simulink model "Morimoto1990_FieldWeakening"  (R2024b)
settings: Solver=FixedStepDiscrete  StartTime=0.0  StopTime=Duration  FixedStep=h  RelTol=1e-3
InitFcn:
  | demoModel=bdroot; demoWorkspace=get_param(demoModel,'ModelWorkspace');
  | demoCases=getVariable(demoWorkspace,'DemoCases');
  | demoCaseName=get_param([demoModel '/Experiment_Settings'],'CaseName');
  | demoSelected=find(strcmp(demoCaseName,{demoCases.name}),1);
  | demoValues=demoCases(demoSelected).variables; demoNames=fieldnames(demoValues);
  | for demoIndex=1:numel(demoNames), assignin(demoWorkspace,demoNames{demoIndex},demoValues.(demoNames{demoIndex})); end
  | clear demoModel demoWorkspace demoCases demoCaseName demoSelected demoValues demoNames demoIndex;
model workspace (MAT data in the model file):
  DemoCases : object (value not decoded)
  SpeedProgram = [0  0; 0.22  900; 0.34  900; 0.95  4200; 1.65  4200]
  UseWeakening = 1
values from neighbouring files (symbols this model uses):
  B = 0.0002    [Morimoto1990_FieldWeakening.sldd]
  BaseCap = 11.4197598 11.4197598 11.4197598 11.4197598 11.4197598 11.4197598 11.4197598 11.4197598 11.4197598 11.4197598 11.4197598 11.4197598 11.4197598 11.4197598 11.4197598 11.4197598 11.4197598 11.4197598 11.4197598 11.4197598 11.4197598 11.4197598 11.4197598 11.4197598 11.4197598 11.4197598 11.4197598 11.4197598 11.4197598 11.4197598 11.4197598 11.4197598 11.4197598 11.4197598 11.4197598 11.4197598 11.4    [Morimoto1990_FieldWeakening.sldd]
  BaseId = -0.0 -0.0 -0.0 -0.0 -0.0 -0.0 -0.0 -0.0 -0.0 -0.0 -0.0 -0.0 -0.0 -0.0 -0.0 -0.0 -0.0 -0.0 -0.0 -0.0 -0.0 -0.0 -0.0 -0.0 -0.0 -0.0 -0.0 -0.0 -0.0 -0.0 -0.0 -0.0 -0.0 -0.0 -0.0 -0.0 -0.0 -0.0 -0.0 -0.0 -0.0 -0.0 -0.0 -0.0 -0.0 -0.0 -0.0 -0.0 -0.0 -0.0 -0.0 -0.0 -0.0 -0.0 -0.0 -0.0 -0.0 -0.0 -0.0 -0.0 -0.0 -0.0 -0.0 -0.0 -0.0 -0.0 -0.0 -0.0 -0.0 -0.0 -0.0 -0.0 -0.0 -0.0 -0.0 -0.0 -0.0 -0.0 -0.0 -0.0    [Morimoto1990_FieldWeakening.sldd]
  BaseIq = 0.0 0.0 0.0 0.0 0.0 0.0 0.0 0.0 0.0 0.0 0.0 0.0 0.0 0.0 0.0 0.0 0.0 0.0 0.0 0.0 0.0 0.0 0.0 0.0 0.0 0.0 0.0 0.0 0.0 0.0 0.0 0.0 0.0 0.0 0.0 0.0 0.0 0.0 0.0 0.0 0.0 0.0 0.0 0.0 0.0 0.0 0.0 0.0 0.0 0.0 0.0 0.0 0.0 0.0 0.0 0.0 0.0 0.0 0.0 0.0 0.0 0.0 0.0 0.0 0.0 0.0 0.0 0.0 0.0 0.0 0.0 0.0 0.0 0.0 0.0 0.0 0.0 0.0 0.0 0.0 0.0 0.0 0.0 0.0 0.0 0.0 0.0 0.0 0.0 0.0 0.0 0.0 0.0 0.0 0.0 0.0 0.0 0.0 0.0 0.0    [Morimoto1990_FieldWeakening.sldd]
  BusReadyRatio = 0.94    [Morimoto1990_FieldWeakening.sldd]
  CurrentBandwidth = 1450.0    [Morimoto1990_FieldWeakening.sldd]
  CurrentKaw = 1500.0    [Morimoto1990_FieldWeakening.sldd]
  EnableThreshold = 0.5    [Morimoto1990_FieldWeakening.sldd]
  Fraction = 0.0 0.025 0.05 0.075 0.1 0.125 0.15 0.175 0.2 0.225 0.25 0.275 0.3 0.325 0.35 0.375 0.4 0.425 0.45 0.475 0.5 0.525 0.55 0.575 0.6 0.625 0.65 0.675 0.7 0.725 0.75 0.775 0.8 0.825 0.85 0.875 0.9 0.925 0.95 0.975 1.0    [Morimoto1990_FieldWeakening.sldd]
  FwCap = 11.4197598 11.4197598 11.4197598 11.4197598 11.4197598 11.4197598 11.4197598 11.4197598 11.4197598 11.4197598 11.4197598 11.4197598 11.4197598 11.4197598 11.4197598 11.4197598 11.4197598 11.4197598 11.4197598 11.4197598 11.4197598 11.4197598 11.4197598 11.4197598 11.4197598 11.4197598 11.4197598 11.4197598 11.4197598 11.4197598 11.4197598 11.4197598 11.4197598 11.4197598 11.4197598 11.4197598 11.4    [Morimoto1990_FieldWeakening.sldd]
  FwId = -0.0 -0.0 -0.0 -0.0 -0.0 -0.0 -0.0 -0.0 -0.0 -0.0 -0.0 -0.0 -0.0 -0.0 -0.0 -0.0 -0.0 -0.0 -0.0 -0.0 -0.0 -0.0 -0.0 -0.0 -0.0 -0.0 -0.0 -0.0 -0.0 -0.0 -0.0 -0.0 -0.0 -0.0 -0.0 -0.0 -0.0 -0.0 -0.0 -0.0 -0.0 -0.0 -0.0 -0.0 -0.0 -0.0 -0.0 -0.0 -0.0 -0.0 -0.0 -0.0 -0.0 -0.0 -0.0 -0.0 -0.0 -0.0 -0.0 -0.0 -0.0 -0.0 -0.0 -0.0 -0.0 -0.0 -0.0 -0.0 -0.0 -0.0 -0.0 -0.0 -0.0 -0.0 -0.0 -0.0 -0.0 -0.0 -0.0 -0.0    [Morimoto1990_FieldWeakening.sldd]
  FwIq = 0.0 0.0 0.0 0.0 0.0 0.0 0.0 0.0 0.0 0.0 0.0 0.0 0.0 0.0 0.0 0.0 0.0 0.0 0.0 0.0 0.0 0.0 0.0 0.0 0.0 0.0 0.0 0.0 0.0 0.0 0.0 0.0 0.0 0.0 0.0 0.0 0.0 0.0 0.0 0.0 0.0 0.0 0.0 0.0 0.0 0.0 0.0 0.0 0.0 0.0 0.0 0.0 0.0 0.0 0.0 0.0 0.0 0.0 0.0 0.0 0.0 0.0 0.0 0.0 0.0 0.0 0.0 0.0 0.0 0.0 0.0 0.0 0.0 0.0 0.0 0.0 0.0 0.0 0.0 0.0 0.0 0.0 0.0 0.0 0.0 0.0 0.0 0.0 0.0 0.0 0.0 0.0 0.0 0.0 0.0 0.0 0.0 0.0 0.0 0.0    [Morimoto1990_FieldWeakening.sldd]
  h = 2.5E-6    [Morimoto1990_FieldWeakening.sldd]
  J = 0.0006    [Morimoto1990_FieldWeakening.sldd]
  Ld = 0.001875    [Morimoto1990_FieldWeakening.sldd]
  Lq = 0.00375    [Morimoto1990_FieldWeakening.sldd]
  Ngrid = 0.0 25.0 50.0 75.0 100.0 125.0 150.0 175.0 200.0 225.0 250.0 275.0 300.0 325.0 350.0 375.0 400.0 425.0 450.0 475.0 500.0 525.0 550.0 575.0 600.0 625.0 650.0 675.0 700.0 725.0 750.0 775.0 800.0 825.0 850.0 875.0 900.0 925.0 950.0 975.0 1000.0 1025.0 1050.0 1075.0 1100.0 1125.0 1150.0 1175.0 1200.0 1225.0 1250.0 1275.0 1300.0 1325.0 1350.0 1375.0 1400.0 1425.0 1450.0 1475.0 1500.0 1525.0 1550.0 1575    [Morimoto1990_FieldWeakening.sldd]
  Pairs = 4.0    [Morimoto1990_FieldWeakening.sldd]
  Psi = 0.045    [Morimoto1990_FieldWeakening.sldd]
  R = 0.065    [Morimoto1990_FieldWeakening.sldd]
  SpeedKaw = 90.0    [Morimoto1990_FieldWeakening.sldd]
  SpeedKi = 1.3    [Morimoto1990_FieldWeakening.sldd]
  SpeedKp = 0.018    [Morimoto1990_FieldWeakening.sldd]
  Ts = 0.0001    [Morimoto1990_FieldWeakening.sldd]
  Vdc = 86.602540378443862    [Morimoto1990_FieldWeakening.sldd]
  VoltageUtilization = 0.98    [Morimoto1990_FieldWeakening.sldd]
(part 2 of 2)

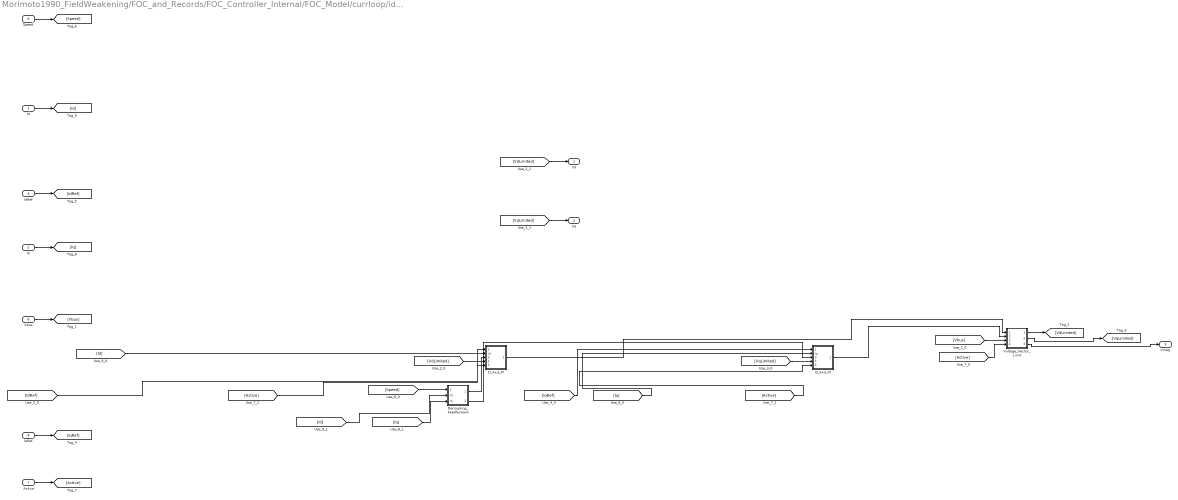
== system Morimoto1990_FieldWeakening/FOC_and_Records/FOC_Controller_Internal/FOC_Model/currloop/idq_Controller ==
  Id : Inport
  Iq : Inport  Port=2
  IdRef : Inport  Port=3
  IqRef : Inport  Port=4
  Speed : Inport  Port=5
  Vbus : Inport  Port=6
  Active : Inport  Port=7
  D_Axis_PI : Subsystem
  Decoupling_Feedforward : Subsystem
  Q_Axis_PI : Subsystem
  Voltage_Vector_Limit : Subsystem
  Vd : Outport
  Vq : Outport  Port=2
  Vmag : Outport  Port=3
  wires:
  [VqLimited] -> Vq/1
  [VdLimited] -> Vd/1
  Vbus/1 -> [Vbus]
  IqRef/1 -> [IqRef]
  IdRef/1 -> [IdRef]
  Speed/1 -> [Speed]
  Active/1 -> [Active]
  Iq/1 -> [Iq]
  Id/1 -> [Id]
  Decoupling_Feedforward/1(VdFF) -> D_Axis_PI/3(VdFF)
  Decoupling_Feedforward/2(VqFF) -> Q_Axis_PI/3(VqFF)
  Voltage_Vector_Limit/2(VqLimited) -> [VqLimited]
  Voltage_Vector_Limit/1(VdLimited) -> [VdLimited]
  Q_Axis_PI/1(VqRaw) -> Voltage_Vector_Limit/2(VqRaw)
  D_Axis_PI/1(VdRaw) -> Voltage_Vector_Limit/1(VdRaw)
  Voltage_Vector_Limit/3(Vmag) -> Vmag/1
  [Vbus] -> Voltage_Vector_Limit/3(Vbus)
  [VdLimited] -> D_Axis_PI/4(VdLimited)
  [VqLimited] -> Q_Axis_PI/4(VqLimited)
  [IqRef] -> Q_Axis_PI/1(IqRef)
  [IdRef] -> D_Axis_PI/1(IdRef)
  [Speed] -> Decoupling_Feedforward/1(Speed)
  [Active] -> Voltage_Vector_Limit/4(Active)
  [Active] -> Q_Axis_PI/5(Active)
  [Active] -> D_Axis_PI/5(Active)
  [Iq] -> Q_Axis_PI/2(Iq)
  [Iq] -> Decoupling_Feedforward/3(Iq)
  [Id] -> D_Axis_PI/2(Id)
  [Id] -> Decoupling_Feedforward/2(Id)

== system Morimoto1990_FieldWeakening/FOC_and_Records/FOC_Controller_Internal/FOC_Model/speedloop/Speed_PI ==
  SpeedRef : Inport
  Active : Inport  Port=2
  TorqueCap : Inport  Port=3
  Speed : Inport  Port=4
  Enabled_torque : Product
  Motoring_only : MinMax  Function=max  Inputs=2
  Next_speed_state : Sum
  Reset_speed_state : Product
  Speed_Ki : Gain  Gain=SpeedKi
  Speed_Kp : Gain  Gain=SpeedKp
  Speed_PI_state : UnitDelay  InitialCondition=single(0)  SampleTime=Ts  HasFrameUpgradeWarning=on
  Speed_antiwindup : Gain  Gain=SpeedKaw
  Speed_error : Sum  Inputs=+-
  Speed_integral_step : Gain  Gain=Ts
  Speed_integrator_input : Sum
  Torque_request : Sum
  Torque_residual : Sum  Inputs=+-
  Torque_upper_limit : MinMax  Inputs=2
  Zero_torque : Constant  Value=0  OutDataTypeStr=single
  TorqueCmd : Outport
  wires:
  Zero_torque/1 -> Motoring_only/2
  Torque_residual/1 -> Speed_antiwindup/1
  Speed_Ki/1 -> Speed_integrator_input/1
  Active/1 -> Reset_speed_state/2, Enabled_torque/2
  Speed_integrator_input/1 -> Speed_integral_step/1
  Torque_request/1 -> Torque_upper_limit/1, Torque_residual/2
  Speed_integral_step/1 -> Next_speed_state/2
  Enabled_torque/1 -> Torque_residual/1, TorqueCmd/1
  Speed_antiwindup/1 -> Speed_integrator_input/2
  SpeedRef/1 -> Speed_error/1
  Torque_upper_limit/1 -> Motoring_only/1
  Reset_speed_state/1 -> Speed_PI_state/1
  Speed_Kp/1 -> Torque_request/1
  Speed_error/1 -> Speed_Ki/1, Speed_Kp/1
  Speed_PI_state/1 -> Next_speed_state/1, Torque_request/2
  TorqueCap/1 -> Torque_upper_limit/2
  Motoring_only/1 -> Enabled_torque/1
  Next_speed_state/1 -> Reset_speed_state/1
  Speed/1 -> Speed_error/2

== system Morimoto1990_FieldWeakening/FOC_and_Records/FOC_Controller_Internal/FOC_Model/speedloop/Torque_Capacity ==
  UseFW : Inport
  Speed : Inport  Port=2
  MTPA_ceiling : Lookup_n-D  NumberOfTableDimensions=1  BreakpointsForDimension1=Ngrid  BreakpointsForDimension3=[5, 7]  Table=BaseCap  ExtrapMethod=Clip  InternalRulePriority=Speed  RndMeth=Simplest
  Select_ceiling : Switch  Criteria=u2 > Threshold  Threshold=0.5  SaturateOnIntegerOverflow=off  InputSameDT=off
  Speed_magnitude : Abs  SaturateOnIntegerOverflow=off
  Weakening_ceiling : Lookup_n-D  NumberOfTableDimensions=1  BreakpointsForDimension1=Ngrid  BreakpointsForDimension3=[5, 7]  Table=FwCap  ExtrapMethod=Clip  InternalRulePriority=Speed  RndMeth=Simplest
  TorqueCap : Outport
  wires:
  MTPA_ceiling/1 -> Select_ceiling/3
  Weakening_ceiling/1 -> Select_ceiling/1
  UseFW/1 -> Select_ceiling/2
  Speed_magnitude/1 -> MTPA_ceiling/1, Weakening_ceiling/1
  Speed/1 -> Speed_magnitude/1
  Select_ceiling/1 -> TorqueCap/1

== system Morimoto1990_FieldWeakening/FOC_and_Records/FOC_Controller_Internal/FOC_Model/speedloop/Torque_Normalization ==
  TorqueCmd : Inport
  TorqueCap : Inport  Port=2
  Minimum_capacity : Constant  Value=0.0001  OutDataTypeStr=single
  Normalized_torque : Product  Inputs=*/
  Safe_capacity : MinMax  Function=max  Inputs=2
  Fraction : Outport
  wires:
  Safe_capacity/1 -> Normalized_torque/2
  Minimum_capacity/1 -> Safe_capacity/2
  Normalized_torque/1 -> Fraction/1
  TorqueCap/1 -> Safe_capacity/1
  TorqueCmd/1 -> Normalized_torque/1

== system Morimoto1990_FieldWeakening/FOC_and_Records/FOC_Controller_Internal/FOC_Model/currloop/Current_Transform/Clarke ==
  Ia : Inport
  Ib : Inport  Port=2
  Ic : Inport  Port=3
  Alpha : Gain  Gain=2/3
  Alpha_sum : Sum  Inputs=+--
  B_minus_C : Sum  Inputs=+-
  Beta : Gain  Gain=1/sqrt(3)
  Half_B : Gain  Gain=0.5
  Half_C : Gain  Gain=0.5
  Ialpha : Outport
  Ibeta : Outport  Port=2
  wires:
  Beta/1 -> Ibeta/1
  B_minus_C/1 -> Beta/1
  Half_C/1 -> Alpha_sum/3
  Ia/1 -> Alpha_sum/1
  Ic/1 -> Half_C/1, B_minus_C/2
  Half_B/1 -> Alpha_sum/2
  Ib/1 -> Half_B/1, B_minus_C/1
  Alpha_sum/1 -> Alpha/1
  Alpha/1 -> Ialpha/1

== system Morimoto1990_FieldWeakening/FOC_and_Records/FOC_Controller_Internal/FOC_Model/currloop/Current_Transform/Park ==
  Ialpha : Inport
  Ibeta : Inport  Port=2
  CosTheta : Inport  Port=3
  SinTheta : Inport  Port=4
  Alpha_cos : Product
  Alpha_sin : Product
  Beta_cos : Product
  Beta_sin : Product
  Park_D : Sum
  Park_Q : Sum  Inputs=+-
  Iq : Outport
  Id : Outport  Port=2
  wires:
  Beta_sin/1 -> Park_D/2
  Ibeta/1 -> Beta_cos/1, Beta_sin/1
  Ialpha/1 -> Alpha_sin/1, Alpha_cos/1
  SinTheta/1 -> Beta_sin/2, Alpha_sin/2
  CosTheta/1 -> Alpha_cos/2, Beta_cos/2
  Alpha_sin/1 -> Park_Q/2
  Beta_cos/1 -> Park_Q/1
  Alpha_cos/1 -> Park_D/1
  Park_D/1 -> Id/1
  Park_Q/1 -> Iq/1

== system Morimoto1990_FieldWeakening/FOC_and_Records/FOC_Controller_Internal/FOC_Model/currloop/Current_Transform/SinCos ==
  Theta : Inport
  Cos_theta : Trigonometry  Operator=cos
  Sin_theta : Trigonometry
  CosTheta : Outport
  SinTheta : Outport  Port=2
  wires:
  Sin_theta/1 -> SinTheta/1
  Theta/1 -> Sin_theta/1, Cos_theta/1
  Cos_theta/1 -> CosTheta/1

== system Morimoto1990_FieldWeakening/FOC_and_Records/FOC_Controller_Internal/FOC_Model/currloop/SVPWM/Angle_Advance ==
  Theta : Inport
  Speed : Inport  Port=2
  Advanced_theta : Sum
  Cos_theta : Trigonometry  Operator=cos
  Half_carrier_advance : Gain  Gain=pi/30*Pairs*Ts/2
  Sin_theta : Trigonometry
  SinTheta : Outport
  CosTheta : Outport  Port=2
  wires:
  Advanced_theta/1 -> Sin_theta/1, Cos_theta/1
  Half_carrier_advance/1 -> Advanced_theta/2
  Cos_theta/1 -> CosTheta/1
  Theta/1 -> Advanced_theta/1
  Sin_theta/1 -> SinTheta/1
  Speed/1 -> Half_carrier_advance/1

== system Morimoto1990_FieldWeakening/FOC_and_Records/FOC_Controller_Internal/FOC_Model/currloop/SVPWM/AntiClarke ==
  Valpha : Inport
  Vbeta : Inport  Port=2
  Beta_sqrt3_2 : Gain  Gain=sqrt(3)/2
  Minus_half_alpha : Gain  Gain=-0.5
  Phase_B : Sum
  Phase_C : Sum  Inputs=+-
  Vb : Outport
  Vc : Outport  Port=2
  wires:
  Beta_sqrt3_2/1 -> Phase_B/2, Phase_C/2
  Valpha/1 -> Minus_half_alpha/1
  Minus_half_alpha/1 -> Phase_B/1, Phase_C/1
  Vbeta/1 -> Beta_sqrt3_2/1
  Phase_C/1 -> Vc/1
  Phase_B/1 -> Vb/1

== system Morimoto1990_FieldWeakening/FOC_and_Records/FOC_Controller_Internal/FOC_Model/currloop/SVPWM/AntiPark ==
  Vd : Inport
  SinTheta : Inport  Port=2
  CosTheta : Inport  Port=3
  Vq : Inport  Port=4
  D_cos : Product
  D_sin : Product
  Inverse_Alpha : Sum  Inputs=+-
  Inverse_Beta : Sum
  Q_cos : Product
  Q_sin : Product
  Valpha : Outport
  Vbeta : Outport  Port=2
  wires:
  Vq/1 -> Q_sin/1, Q_cos/1
  Q_cos/1 -> Inverse_Beta/2
  Q_sin/1 -> Inverse_Alpha/2
  Vd/1 -> D_sin/1, D_cos/1
  D_sin/1 -> Inverse_Beta/1
  SinTheta/1 -> Q_sin/2, D_sin/2
  Inverse_Beta/1 -> Vbeta/1
  D_cos/1 -> Inverse_Alpha/1
  CosTheta/1 -> Q_cos/2, D_cos/2
  Inverse_Alpha/1 -> Valpha/1

== system Morimoto1990_FieldWeakening/FOC_and_Records/FOC_Controller_Internal/FOC_Model/currloop/SVPWM/Common_Mode ==
  Vb : Inport
  Valpha : Inport  Port=2
  Vc : Inport  Port=3
  Extrema_sum : Sum
  Negative_common_mode : Gain  Gain=-0.5
  Phase_max : MinMax  Function=max  Inputs=3
  Phase_min : MinMax  Inputs=3
  Voffset : Outport
  wires:
  Extrema_sum/1 -> Negative_common_mode/1
  Vc/1 -> Phase_min/3, Phase_max/3
  Valpha/1 -> Phase_min/1, Phase_max/1
  Vb/1 -> Phase_max/2, Phase_min/2
  Phase_min/1 -> Extrema_sum/2
  Phase_max/1 -> Extrema_sum/1
  Negative_common_mode/1 -> Voffset/1

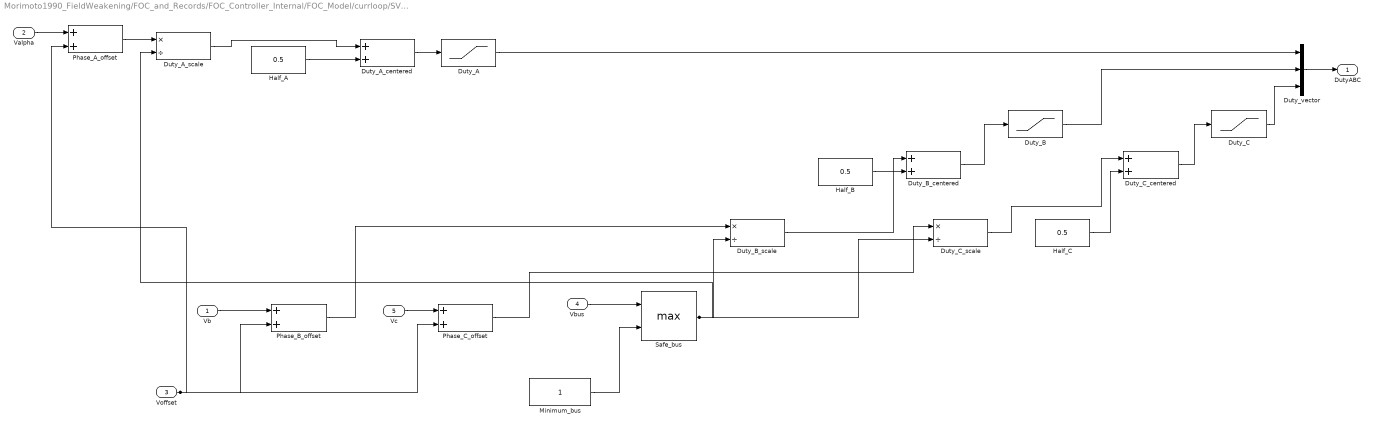
== system Morimoto1990_FieldWeakening/FOC_and_Records/FOC_Controller_Internal/FOC_Model/currloop/SVPWM/Duty_Normalization ==
  Vb : Inport
  Valpha : Inport  Port=2
  Voffset : Inport  Port=3
  Vbus : Inport  Port=4
  Vc : Inport  Port=5
  Duty_A : Saturate  UpperLimit=0.99  LowerLimit=0.01
  Duty_A_centered : Sum
  Duty_A_scale : Product  Inputs=*/
  Duty_B : Saturate  UpperLimit=0.99  LowerLimit=0.01
  Duty_B_centered : Sum
  Duty_B_scale : Product  Inputs=*/
  Duty_C : Saturate  UpperLimit=0.99  LowerLimit=0.01
  Duty_C_centered : Sum
  Duty_C_scale : Product  Inputs=*/
  Duty_vector : Mux  Inputs=3
  Half_A : Constant  Value=0.5  OutDataTypeStr=single
  Half_B : Constant  Value=0.5  OutDataTypeStr=single
  Half_C : Constant  Value=0.5  OutDataTypeStr=single
  Minimum_bus : Constant  OutDataTypeStr=single
  Phase_A_offset : Sum
  Phase_B_offset : Sum
  Phase_C_offset : Sum
  Safe_bus : MinMax  Function=max  Inputs=2
  DutyABC : Outport
  wires:
  Half_C/1 -> Duty_C_centered/2
  Safe_bus/1 -> Duty_A_scale/2, Duty_B_scale/2, Duty_C_scale/2
  Duty_A_centered/1 -> Duty_A/1
  Half_A/1 -> Duty_A_centered/2
  Phase_B_offset/1 -> Duty_B_scale/1
  Duty_A_scale/1 -> Duty_A_centered/1
  Voffset/1 -> Phase_B_offset/2, Phase_C_offset/2, Phase_A_offset/2
  Duty_C_centered/1 -> Duty_C/1
  Phase_A_offset/1 -> Duty_A_scale/1
  Vb/1 -> Phase_B_offset/1
  Minimum_bus/1 -> Safe_bus/2
  Phase_C_offset/1 -> Duty_C_scale/1
  Duty_B_centered/1 -> Duty_B/1
  Duty_B/1 -> Duty_vector/2
  Duty_B_scale/1 -> Duty_B_centered/1
  Duty_C/1 -> Duty_vector/3
  Half_B/1 -> Duty_B_centered/2
  Duty_C_scale/1 -> Duty_C_centered/1
  Duty_A/1 -> Duty_vector/1
  Vc/1 -> Phase_C_offset/1
  Duty_vector/1 -> DutyABC/1
  Vbus/1 -> Safe_bus/1
  Valpha/1 -> Phase_A_offset/1

== system Morimoto1990_FieldWeakening/FOC_and_Records/FOC_Controller_Internal/FOC_Model/currloop/idq_Controller/D_Axis_PI ==
  IdRef : Inport
  Id : Inport  Port=2
  VdFF : Inport  Port=3
  VdLimited : Inport  Port=4
  Active : Inport  Port=5
  Id_Integral_increment : Gain  Gain=Ts
  Id_Integral_input : Sum
  Id_Ki : Gain  Gain=R*CurrentBandwidth
  Id_Kp : Gain  Gain=Ld*CurrentBandwidth
  Id_Next_integral : Sum
  Id_PI_state : UnitDelay  InitialCondition=single(0)  SampleTime=Ts  HasFrameUpgradeWarning=on
  Id_Reset_integral : Product
  Id_Voltage_residual : Sum  Inputs=+-
  Id_antiwindup : Gain  Gain=CurrentKaw
  Id_error : Sum  Inputs=+-
  Vd_unsaturated : Sum  Inputs=+++
  VdRaw : Outport
  wires:
  Id_PI_state/1 -> Vd_unsaturated/2, Id_Next_integral/1
  Id_Integral_input/1 -> Id_Integral_increment/1
  Vd_unsaturated/1 -> Id_Voltage_residual/2, VdRaw/1
  Active/1 -> Id_Reset_integral/2
  Id_error/1 -> Id_Ki/1, Id_Kp/1
  Id_antiwindup/1 -> Id_Integral_input/1
  Id_Ki/1 -> Id_Integral_input/2
  VdLimited/1 -> Id_Voltage_residual/1
  Id_Reset_integral/1 -> Id_PI_state/1
  Id_Voltage_residual/1 -> Id_antiwindup/1
  Id_Integral_increment/1 -> Id_Next_integral/2
  Id_Kp/1 -> Vd_unsaturated/3
  Id_Next_integral/1 -> Id_Reset_integral/1
  VdFF/1 -> Vd_unsaturated/1
  IdRef/1 -> Id_error/1
  Id/1 -> Id_error/2

== system Morimoto1990_FieldWeakening/FOC_and_Records/FOC_Controller_Internal/FOC_Model/currloop/idq_Controller/Decoupling_Feedforward ==
  Speed : Inport
  Id : Inport  Port=2
  Iq : Inport  Port=3
  D_axis_flux : Sum
  D_inductance_flux : Gain  Gain=Ld
  Electrical_speed : Gain  Gain=pi/30*Pairs
  Minus_q_flux : Gain  Gain=-Lq
  PM_flux : Constant  Value=Psi  OutDataTypeStr=single
  d_axis_feedforward : Product
  q_axis_feedforward : Product
  VdFF : Outport
  VqFF : Outport  Port=2
  wires:
  Id/1 -> D_inductance_flux/1
  Minus_q_flux/1 -> d_axis_feedforward/1
  PM_flux/1 -> D_axis_flux/2
  Electrical_speed/1 -> d_axis_feedforward/2, q_axis_feedforward/2
  d_axis_feedforward/1 -> VdFF/1
  D_inductance_flux/1 -> D_axis_flux/1
  Iq/1 -> Minus_q_flux/1
  D_axis_flux/1 -> q_axis_feedforward/1
  Speed/1 -> Electrical_speed/1
  q_axis_feedforward/1 -> VqFF/1

== system Morimoto1990_FieldWeakening/FOC_and_Records/FOC_Controller_Internal/FOC_Model/currloop/idq_Controller/Q_Axis_PI ==
  IqRef : Inport
  Iq : Inport  Port=2
  VqFF : Inport  Port=3
  VqLimited : Inport  Port=4
  Active : Inport  Port=5
  Iq_Integral_increment : Gain  Gain=Ts
  Iq_Integral_input : Sum
  Iq_Ki : Gain  Gain=R*CurrentBandwidth
  Iq_Kp : Gain  Gain=Lq*CurrentBandwidth
  Iq_Next_integral : Sum
  Iq_PI_state : UnitDelay  InitialCondition=single(0)  SampleTime=Ts  HasFrameUpgradeWarning=on
  Iq_Reset_integral : Product
  Iq_Voltage_residual : Sum  Inputs=+-
  Iq_antiwindup : Gain  Gain=CurrentKaw
  Iq_error : Sum  Inputs=+-
  Vq_unsaturated : Sum  Inputs=+++
  VqRaw : Outport
  wires:
  Iq_Integral_increment/1 -> Iq_Next_integral/2
  Iq_error/1 -> Iq_Ki/1, Iq_Kp/1
  Iq_antiwindup/1 -> Iq_Integral_input/1
  Iq_Kp/1 -> Vq_unsaturated/3
  Iq_Ki/1 -> Iq_Integral_input/2
  Vq_unsaturated/1 -> VqRaw/1, Iq_Voltage_residual/2
  Iq_Reset_integral/1 -> Iq_PI_state/1
  Iq_Next_integral/1 -> Iq_Reset_integral/1
  Iq_PI_state/1 -> Vq_unsaturated/2, Iq_Next_integral/1
  Iq_Integral_input/1 -> Iq_Integral_increment/1
  Iq_Voltage_residual/1 -> Iq_antiwindup/1
  VqFF/1 -> Vq_unsaturated/1
  Iq/1 -> Iq_error/2
  IqRef/1 -> Iq_error/1
  Active/1 -> Iq_Reset_integral/2
  VqLimited/1 -> Iq_Voltage_residual/1

== system Morimoto1990_FieldWeakening/FOC_and_Records/FOC_Controller_Internal/FOC_Model/currloop/idq_Controller/Voltage_Vector_Limit ==
  VdRaw : Inport
  VqRaw : Inport  Port=2
  Vbus : Inport  Port=3
  Active : Inport  Port=4
  Enabled_voltage_scale : Product
  Limited_Vd : Product
  Limited_Vq : Product
  Limited_magnitude : Product
  Linear_SVPWM_limit : Gain  Gain=VoltageUtilization/sqrt(3)
  Minimum_magnitude : Constant  Value=0.001  OutDataTypeStr=single
  Safe_magnitude : MinMax  Function=max  Inputs=2
  Unity_scale : Constant  OutDataTypeStr=single
  Vd_squared : Product
  Vector_limiter : MinMax  Inputs=2
  Voltage_circle_ratio : Product  Inputs=*/
  Voltage_request : Sqrt
  Voltage_squared : Sum
  Vq_squared : Product
  VdLimited : Outport
  VqLimited : Outport  Port=2
  Vmag : Outport  Port=3
  wires:
  Voltage_squared/1 -> Voltage_request/1
  Enabled_voltage_scale/1 -> Limited_Vd/1, Limited_Vq/1, Limited_magnitude/2
  Safe_magnitude/1 -> Voltage_circle_ratio/2
  VqRaw/1 -> Limited_Vq/2, Vq_squared/2, Vq_squared/1
  VdRaw/1 -> Limited_Vd/2, Vd_squared/1, Vd_squared/2
  Minimum_magnitude/1 -> Safe_magnitude/2
  Voltage_request/1 -> Limited_magnitude/1, Safe_magnitude/1
  Vq_squared/1 -> Voltage_squared/2
  Voltage_circle_ratio/1 -> Vector_limiter/1
  Unity_scale/1 -> Vector_limiter/2
  Vbus/1 -> Linear_SVPWM_limit/1
  Vd_squared/1 -> Voltage_squared/1
  Vector_limiter/1 -> Enabled_voltage_scale/1
  Linear_SVPWM_limit/1 -> Voltage_circle_ratio/1
  Limited_magnitude/1 -> Vmag/1
  Limited_Vd/1 -> VdLimited/1
  Active/1 -> Enabled_voltage_scale/2
  Limited_Vq/1 -> VqLimited/1
